simulink model "ACFT11_a_121_flatearth_backup"  (R2026a)
settings: Solver=ode15s  StopTime=10  FixedStep=0.01  MaxStep=0.05  MinStep=1e-4  AbsTol=1e-4
model workspace (MAT data in the model file):
  op11 : opcond.OperatingPoint (value not decoded)
  op_trim1 : opcond.OperatingReport (value not decoded)
  op_trim12 : opcond.OperatingReport (value not decoded)
  op_trim15 : opcond.OperatingReport (value not decoded)
  op_trim16 : opcond.OperatingReport (value not decoded)
  op_trim17 : opcond.OperatingReport (value not decoded)
  op_trim18 : opcond.OperatingReport (value not decoded)
  op_trim2 : opcond.OperatingReport (value not decoded)
  op_trim20 : opcond.OperatingReport (value not decoded)
  op_trim21 : opcond.OperatingReport (value not decoded)
  op_trim22 : opcond.OperatingReport (value not decoded)
  op_trim23 : opcond.OperatingReport (value not decoded)
  op_trim24 : opcond.OperatingReport (value not decoded)
  op_trim25 : opcond.OperatingReport (value not decoded)
  op_trim29 : opcond.OperatingReport (value not decoded)
  op_trim3 : opcond.OperatingReport (value not decoded)
  op_trim30 : opcond.OperatingReport (value not decoded)
  op_trim4 : opcond.OperatingReport (value not decoded)
  op_trim40 : opcond.OperatingReport (value not decoded)
  op_trim42 : opcond.OperatingReport (value not decoded)
  op_trim5 : opcond.OperatingReport (value not decoded)
  op_trim50 : opcond.OperatingReport (value not decoded)
  op_trim7 : opcond.OperatingReport (value not decoded)
  op_trim9 : opcond.OperatingReport (value not decoded)
values from neighbouring files (symbols this model uses):
  b = min(1, 2*(1-frac))    [export_kml.m]    (also in flight_hud.m = chaseBack; inertiatensor62.m = 9.05; setup_bfl_analysis.m = 9.05; setup_fcs_sim.m = 9.05)
  c = bar_colors{min(k,numel(bar_colors))}    [analyze_bfl.m]    (also in ecef_eom_fcn.m = w_eb_b(3); inertiatensor62.m = 15.55; optimize_indi_gains.m = 15.55; restore_normal_fcs.m = 15.55)
  CL_AlphaDot = 0    [inertiatensor62.m]    (also in setup_bfl_analysis.m; setup_fcs_sim.m; setup_takeoff_fcs.m)
  Cm_AlphaDot = 0    [inertiatensor62.m]    (also in setup_bfl_analysis.m; setup_fcs_sim.m; setup_takeoff_fcs.m)
  F = convhull(pts)    [Visualization_Takeoff2.m]    (also in attitude_ribbon.m = {[1 2 3],[1 4 2],[1 4 3],[4 5 1]})
  FCS_aerospike_thrust = 250000.0    (= 250000)    [fcs_params.m]
  FCS_alpha_max = 16.0    (= 16)    [fcs_params.m]
  FCS_bank_max = 35.0    (= 35)    [fcs_params.m]
  FCS_da_max = 20.0    (= 20)    [fcs_params.m]
  FCS_de_max = 25.0    (= 25)    [fcs_params.m]
  FCS_dr_max = 25.0    (= 25)    [fcs_params.m]
  FCS_dt = 0.01    [fcs_params.m]
  FCS_g = 9.80665    [fcs_params.m]
  FCS_Gmin_p = 0.02    [fcs_params.m]
  FCS_Gmin_q = 0.02    [fcs_params.m]
  FCS_Gmin_r = 0.01    [fcs_params.m]
  FCS_h_gnd = 2.24    [fcs_params.m]
  FCS_hdot_max = 30.0    (= 30)    [fcs_params.m]
  FCS_hdot_td = 0.3    [fcs_params.m]
  FCS_Kalpha = 3.0    (= 3)    [fcs_params.m]
  FCS_Kalpha_lim = 2.0    (= 2)    [fcs_params.m]
  FCS_Kbeta = 2.0    (= 2)    [fcs_params.m]
  FCS_Kflare = 1.0    (= 1)    [fcs_params.m]
  FCS_Kgamma = 1.5    [fcs_params.m]
  FCS_Kh = 0.10    (= 0.1)    [fcs_params.m]
  FCS_Knz = 20.0    (= 20)    [fcs_params.m]
  FCS_Kp = 6.0    (= 6)    [fcs_params.m]
  FCS_Kphi = 3.0    (= 3)    [fcs_params.m]
  FCS_Kq = 5.0    (= 5)    [fcs_params.m]
  FCS_Kr = 4.0    (= 4)    [fcs_params.m]
  FCS_Ktheta = 2.0    (= 2)    [fcs_params.m]
  FCS_link_timeout = 1.0    (= 1)    [fcs_params.m]
  FCS_MODE_AUTO = 0    [fcs_params.m]
  FCS_Nfilt = 20.0    (= 20)    [fcs_params.m]
  FCS_Nz_max = 3.0    (= 3)    [fcs_params.m]
  FCS_Nz_min = -1.0    (= -1)    [fcs_params.m]
  FCS_p_max = 40.0    (= 40)    [fcs_params.m]
  FCS_q_max = 15.0    (= 15)    [fcs_params.m]
  FCS_qbar_hi = 6000.0    (= 6000)    [fcs_params.m]
  FCS_qbar_lo = 1000.0    (= 1000)    [fcs_params.m]
  FCS_r_max = 15.0    (= 15)    [fcs_params.m]
  FCS_relight_M_hi = 2.0    (= 2)    [fcs_params.m]
  FCS_relight_M_lo = 0.35    [fcs_params.m]
  FCS_relight_qbar = 3000.0    (= 3000)    [fcs_params.m]
  FCS_stick_detent = 0.03    [fcs_params.m]
  FCS_stick_p_scale = 60.0    (= 60)    [fcs_params.m]
  FCS_stick_q_scale = 15.0    (= 15)    [fcs_params.m]
  FCS_tau_flare = 3.0    (= 3)    [fcs_params.m]
  FCS_TECS_Kep = 0.25    [fcs_params.m]
  FCS_TECS_Ktp = 0.30    (= 0.3)    [fcs_params.m]
  FCS_theta_climb = 12.0    (= 12)    [fcs_params.m]
  FCS_theta_max = 30.0    (= 30)    [fcs_params.m]
  FCS_theta_min = -20.0    (= -20)    [fcs_params.m]
  FCS_theta_trim = 0.0    (= 0)    [fcs_params.m]
  FCS_thr_max = 1.0    (= 1)    [fcs_params.m]
  FCS_thr_min = 0.0    (= 0)    [fcs_params.m]
  FCS_thr_trim = 0.50    (= 0.5)    [fcs_params.m]
  FCS_V_rotate = 94.0    (= 94)    [fcs_params.m]
  FCS_Vmin = 60.0    (= 60)    [fcs_params.m]
  FF_rates = [0.0,              2.5,              5.0,             73.0,             78.0,              0.5]    [fcs_params.m]
  g = @(n,d) i_basevar(n,d)    [analyze_control_authority.m]    (also in export_kml.m = 1 - abs(2*frac-1); inertiatensor62.m = 9.80665; setup_bfl_analysis.m = 9.80665; setup_fcs_sim.m = 9.80665)
  GS_Gp_tab = Cl_da * (S*b/Ixx)    [setup_gschedule.m]
  GS_Gq_tab = Cm_de * (S*c/Iyy)    [setup_gschedule.m]
  GS_Gr_tab = Cn_dr * (S*b/Izz)    [setup_gschedule.m]
  MASS_fuel_total = MASS_full - MASS_empty - MASS_orbiter    (= 14700)    [fcs_params.m]
  q = q/norm(q)    [build_ecef_x0.m]    (also in ecef_eom_fcn.m = state(7:10); ecef_out_fcn.m = state(7:10); setup_ecef.m; test_ecef_eom.m = state(7:10))
  r = [0;diff(xc)]/0.1    [analyze_control_authority.m]    (also in ecef_eom_fcn.m = sqrt(r_e(1)^2+r_e(2)^2+r_e(3)^2); ecef_weight_body.m = sqrt(x^2 + y^2 + z^2); export_kml.m = min(1, 2*frac); test_ecef_eom.m = sqrt(r_e(1)^2+r_e(2)^2+r_e(3)^2))
  S = {'\delta_e',DE,lim.de,'b'; '\delta_a',DA,lim.da,[0 .6 0]; '\delta_r',DR,lim.dr,[.85 .3 .1]}    [analyze_control_authority.m]    (also in attitude_ribbon.m = load(char(src)); build_ecef_x0.m = sqrt(1+C(3,3)-C(1,1)-C(2,2))*2; export_kml.m = load(char(src)); flight_hud.m = load(char(src)))
  s = A.surfaces(i)    [analyze_control_authority.m]    (also in setup_propulsion.m = [s, sprintf(')
  y_cg = 0    [inertiatensor62.m]    (also in setup_bfl_analysis.m; setup_fcs_sim.m; setup_takeoff_fcs.m)
  z_cg = 0.0    (= 0)    [inertiatensor62.m]    (also in setup_bfl_analysis.m; setup_fcs_sim.m; setup_takeoff_fcs.m)
undefined symbols (not defined in the file or in its folder): deg, DiscIntNeverNeededParam, EqM, GS_alpha_cl, GS_alpha_cm, GS_alpha_cn, GS_mach_cl, GS_mach_cm, GS_mach_cn, MIL, Moderate, rad
libraries: aerolibconvert2 x21, simulink x7, aerolibfltsims x3, aerolibwind2 x3, aerolibanim x1, aerolibatmos2 x1, shareddyn x1, aerolibobsolete x1
(part 4 of 4)

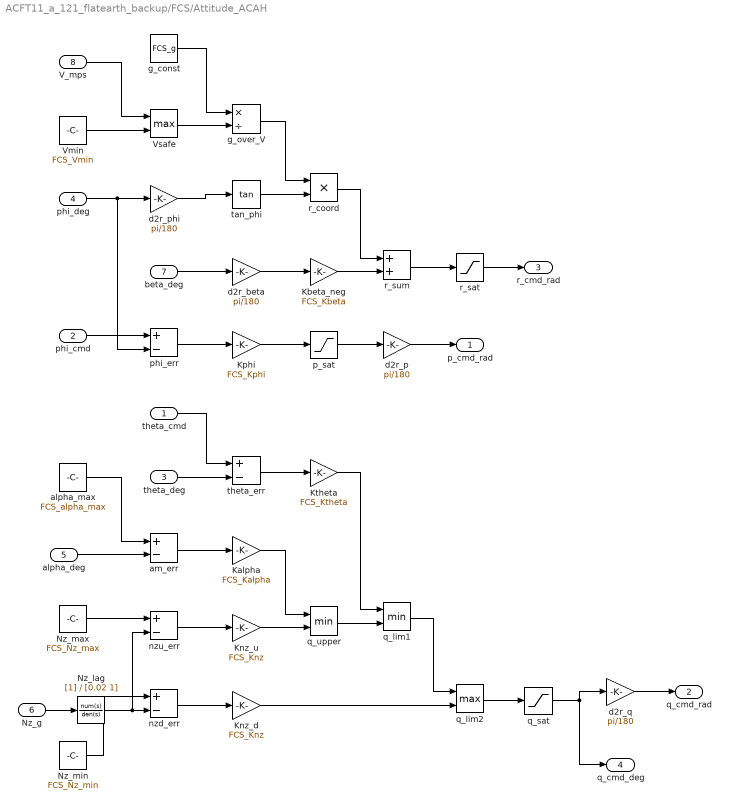
== system ACFT11_a_121_flatearth_backup/FCS/Attitude_ACAH ==
  theta_cmd : Inport
  phi_cmd : Inport  Port=2
  theta_deg : Inport  Port=3
  phi_deg : Inport  Port=4
  alpha_deg : Inport  Port=5
  Nz_g : Inport  Port=6
  beta_deg : Inport  Port=7
  V_mps : Inport  Port=8
  Kalpha : Gain  Gain=FCS_Kalpha
  Kbeta_neg : Gain  Gain=FCS_Kbeta
  Knz_d : Gain  Gain=FCS_Knz
  Knz_u : Gain  Gain=FCS_Knz
  Kphi : Gain  Gain=FCS_Kphi
  Ktheta : Gain  Gain=FCS_Ktheta
  Nz_lag : TransferFcn  Denominator=[0.02 1]
  Nz_max : Constant  Value=FCS_Nz_max
  Nz_min : Constant  Value=FCS_Nz_min
  Vmin : Constant  Value=FCS_Vmin
  Vsafe : MinMax  Function=max  Inputs=2
  alpha_max : Constant  Value=FCS_alpha_max
  am_err : Sum  Inputs=+-
  d2r_beta : Gain  Gain=pi/180
  d2r_p : Gain  Gain=pi/180
  d2r_phi : Gain  Gain=pi/180
  d2r_q : Gain  Gain=pi/180
  g_const : Constant  Value=FCS_g
  g_over_V : Product  Inputs=*/
  nzd_err : Sum  Inputs=+-
  nzu_err : Sum  Inputs=+-
  p_sat : Saturate  UpperLimit=FCS_p_max  LowerLimit=-FCS_p_max
  phi_err : Sum  Inputs=+-
  q_lim1 : MinMax  Inputs=2
  q_lim2 : MinMax  Function=max  Inputs=2
  q_sat : Saturate  UpperLimit=FCS_q_max  LowerLimit=-FCS_q_max
  q_upper : MinMax  Inputs=2
  r_coord : Product  Inputs=**
  r_sat : Saturate  UpperLimit=FCS_r_max*pi/180  LowerLimit=-FCS_r_max*pi/180
  r_sum : Sum
  tan_phi : Trigonometry  Operator=tan
  theta_err : Sum  Inputs=+-
  p_cmd_rad : Outport
  q_cmd_rad : Outport  Port=2
  r_cmd_rad : Outport  Port=3
  q_cmd_deg : Outport  Port=4
  wires:
  r_sat/1 -> r_cmd_rad/1
  r_sum/1 -> r_sat/1
  Kbeta_neg/1 -> r_sum/2
  r_coord/1 -> r_sum/1
  d2r_beta/1 -> Kbeta_neg/1
  beta_deg/1 -> d2r_beta/1
  tan_phi/1 -> r_coord/2
  g_over_V/1 -> r_coord/1
  Vsafe/1 -> g_over_V/2
  g_const/1 -> g_over_V/1
  Vmin/1 -> Vsafe/2
  V_mps/1 -> Vsafe/1
  d2r_phi/1 -> tan_phi/1
  d2r_p/1 -> p_cmd_rad/1
  p_sat/1 -> d2r_p/1
  Kphi/1 -> p_sat/1
  phi_err/1 -> Kphi/1
  phi_deg/1 -> phi_err/2, d2r_phi/1
  phi_cmd/1 -> phi_err/1
  d2r_q/1 -> q_cmd_rad/1
  q_sat/1 -> q_cmd_deg/1, d2r_q/1
  q_lim2/1 -> q_sat/1
  Knz_d/1 -> q_lim2/2
  q_lim1/1 -> q_lim2/1
  q_upper/1 -> q_lim1/2
  Ktheta/1 -> q_lim1/1
  Knz_u/1 -> q_upper/2
  Kalpha/1 -> q_upper/1
  nzd_err/1 -> Knz_d/1
  Nz_min/1 -> nzd_err/1
  nzu_err/1 -> Knz_u/1
  Nz_max/1 -> nzu_err/1
  am_err/1 -> Kalpha/1
  alpha_deg/1 -> am_err/2
  alpha_max/1 -> am_err/1
  theta_err/1 -> Ktheta/1
  theta_deg/1 -> theta_err/2
  theta_cmd/1 -> theta_err/1
  Nz_g/1 -> Nz_lag/1
  Nz_lag/1 -> nzu_err/2, nzd_err/2

== system ACFT11_a_121_flatearth_backup/FCS/HeadingHold ==
  track : Inport
  psi_cmd : Inport  Port=2
  V : Inport  Port=3
  qbar : Inport  Port=4
  L1law : MATLAB Function  TreatAsAtomicUnit=on
  bank_sat : Saturate  UpperLimit=FCS_bank_max  LowerLimit=-FCS_bank_max
  phi_cmd : Outport
  wires:
  L1law/1(phi) -> bank_sat/1
  V/1 -> L1law/3(V)
  track/1 -> L1law/2(track)
  psi_cmd/1 -> L1law/1(psi_cmd)
  bank_sat/1 -> phi_cmd/1
  qbar/1 -> L1law/4(qbar)

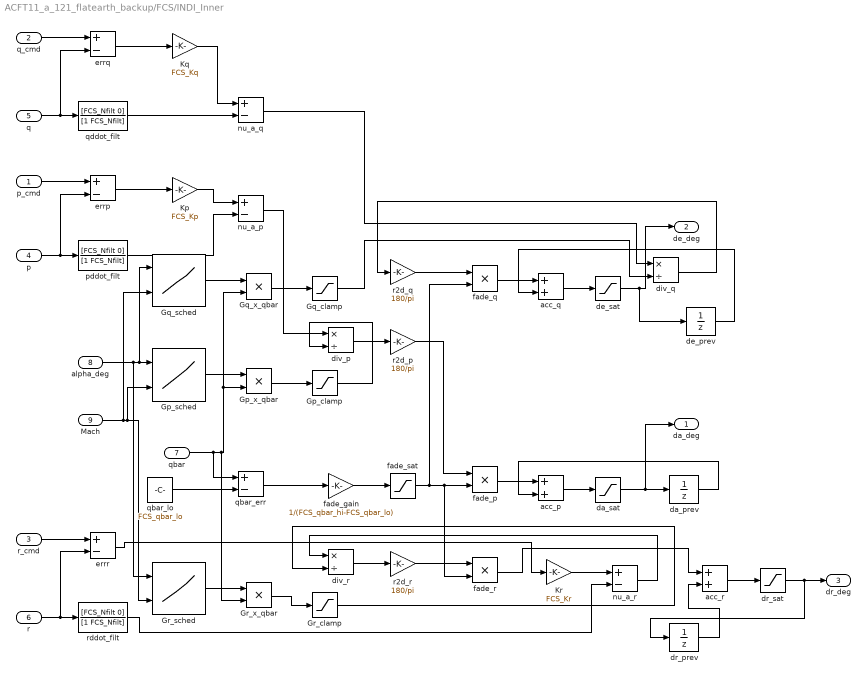
== system ACFT11_a_121_flatearth_backup/FCS/INDI_Inner ==
  p_cmd : Inport
  q_cmd : Inport  Port=2
  r_cmd : Inport  Port=3
  p : Inport  Port=4
  q : Inport  Port=5
  r : Inport  Port=6
  qbar : Inport  Port=7
  alpha_deg : Inport  Port=8
  Mach : Inport  Port=9
  Gp_clamp : Saturate  UpperLimit=-FCS_Gmin_p  LowerLimit=-1e6
  Gp_sched : Lookup_n-D  BreakpointsForDimension1=GS_alpha_cl  BreakpointsForDimension2=GS_mach_cl  Table=GS_Gp_tab  ExtrapMethod=Clip  InternalRulePriority=Speed  RndMeth=Simplest
      settings: InputPortMap=u0,u1
  Gp_x_qbar : Product
  Gq_clamp : Saturate  UpperLimit=-FCS_Gmin_q  LowerLimit=-1e6
  Gq_sched : Lookup_n-D  BreakpointsForDimension1=GS_alpha_cm  BreakpointsForDimension2=GS_mach_cm  Table=GS_Gq_tab  ExtrapMethod=Clip  InternalRulePriority=Speed  RndMeth=Simplest
      settings: InputPortMap=u0,u1
  Gq_x_qbar : Product
  Gr_clamp : Saturate  UpperLimit=-FCS_Gmin_r  LowerLimit=-1e6
  Gr_sched : Lookup_n-D  BreakpointsForDimension1=GS_alpha_cn  BreakpointsForDimension2=GS_mach_cn  Table=GS_Gr_tab  ExtrapMethod=Clip  InternalRulePriority=Speed  RndMeth=Simplest
      settings: InputPortMap=u0,u1
  Gr_x_qbar : Product
  Kp : Gain  Gain=FCS_Kp
  Kq : Gain  Gain=FCS_Kq
  Kr : Gain  Gain=FCS_Kr
  acc_p : Sum
  acc_q : Sum
  acc_r : Sum
  da_prev : UnitDelay  SampleTime=FCS_dt
  da_sat : Saturate  UpperLimit=FCS_da_max  LowerLimit=-FCS_da_max
  de_prev : UnitDelay  SampleTime=FCS_dt
  de_sat : Saturate  UpperLimit=FCS_de_max  LowerLimit=-FCS_de_max
  div_p : Product  Inputs=*/
  div_q : Product  Inputs=*/
  div_r : Product  Inputs=*/
  dr_prev : UnitDelay  SampleTime=FCS_dt
  dr_sat : Saturate  UpperLimit=FCS_dr_max  LowerLimit=-FCS_dr_max
  errp : Sum  Inputs=+-
  errq : Sum  Inputs=+-
  errr : Sum  Inputs=+-
  fade_gain : Gain  Gain=1/(FCS_qbar_hi-FCS_qbar_lo)
  fade_p : Product  Inputs=**
  fade_q : Product  Inputs=**
  fade_r : Product  Inputs=**
  fade_sat : Saturate  UpperLimit=1  LowerLimit=0
  nu_a_p : Sum  Inputs=+-
  nu_a_q : Sum  Inputs=+-
  nu_a_r : Sum  Inputs=+-
  pddot_filt : TransferFcn  Numerator=[FCS_Nfilt 0]  Denominator=[1 FCS_Nfilt]
  qbar_err : Sum  Inputs=+-
  qbar_lo : Constant  Value=FCS_qbar_lo
  qddot_filt : TransferFcn  Numerator=[FCS_Nfilt 0]  Denominator=[1 FCS_Nfilt]
  r2d_p : Gain  Gain=180/pi
  r2d_q : Gain  Gain=180/pi
  r2d_r : Gain  Gain=180/pi
  rddot_filt : TransferFcn  Numerator=[FCS_Nfilt 0]  Denominator=[1 FCS_Nfilt]
  da_deg : Outport
  de_deg : Outport  Port=2
  dr_deg : Outport  Port=3
  wires:
  r2d_r/1 -> fade_r/1
  fade_p/1 -> acc_p/1
  r2d_p/1 -> fade_p/1
  fade_q/1 -> acc_q/1
  fade_sat/1 -> fade_p/2, fade_r/2, fade_q/2
  r2d_q/1 -> fade_q/1
  fade_gain/1 -> fade_sat/1
  qbar_err/1 -> fade_gain/1
  qbar_lo/1 -> qbar_err/2
  da_sat/1 -> da_prev/1, da_deg/1
  acc_p/1 -> da_sat/1
  da_prev/1 -> acc_p/2
  div_p/1 -> r2d_p/1
  nu_a_p/1 -> div_p/1
  pddot_filt/1 -> nu_a_p/2
  Kp/1 -> nu_a_p/1
  errp/1 -> Kp/1
  p/1 -> errp/2, pddot_filt/1
  p_cmd/1 -> errp/1
  qddot_filt/1 -> nu_a_q/2
  Kq/1 -> nu_a_q/1
  errq/1 -> Kq/1
  q/1 -> errq/2, qddot_filt/1
  q_cmd/1 -> errq/1
  acc_q/1 -> de_sat/1
  r_cmd/1 -> errr/1
  r/1 -> rddot_filt/1, errr/2
  div_r/1 -> r2d_r/1
  Gr_x_qbar/1 -> Gr_clamp/1
  Gr_sched/1 -> Gr_x_qbar/1
  Gp_x_qbar/1 -> Gp_clamp/1
  Gp_sched/1 -> Gp_x_qbar/1
  Gq_x_qbar/1 -> Gq_clamp/1
  Gq_sched/1 -> Gq_x_qbar/1
  Mach/1 -> Gr_sched/2, Gp_sched/2, Gq_sched/2
  alpha_deg/1 -> Gq_sched/1, Gp_sched/1, Gr_sched/1
  dr_sat/1 -> dr_prev/1, dr_deg/1
  acc_r/1 -> dr_sat/1
  dr_prev/1 -> acc_r/2
  Gr_clamp/1 -> div_r/2
  nu_a_r/1 -> div_r/1
  rddot_filt/1 -> nu_a_r/2
  Kr/1 -> nu_a_r/1
  errr/1 -> Kr/1
  de_sat/1 -> de_prev/1, de_deg/1
  Gq_clamp/1 -> div_q/2
  qbar/1 -> Gp_x_qbar/2, Gq_x_qbar/2, Gr_x_qbar/2, qbar_err/1
  nu_a_q/1 -> div_q/1
  div_q/1 -> r2d_q/1
  de_prev/1 -> acc_q/2
  Gp_clamp/1 -> div_p/2
  fade_r/1 -> acc_r/1

== system ACFT11_a_121_flatearth_backup/FCS/ModeManager ==
  RC_mode : Inport
  RC_cmd_age : Inport  Port=2
  theta_TECS : Inport  Port=3
  theta_ref : Inport  Port=4
  phi_hdg : Inport  Port=5
  phi_ref : Inport  Port=6
  AUTO : Constant  Value=FCS_MODE_AUTO
  link_lost : simulink/Logic and Bit Operations/Compare To Constant  relop=>  const=FCS_link_timeout  OutDataTypeStr=boolean
  mode_sw : Switch  Threshold=0.5  SaturateOnIntegerOverflow=off  InputSameDT=off
  phi_sw : Switch  Threshold=0.5  SaturateOnIntegerOverflow=off  InputSameDT=off
  theta_sw : Switch  Threshold=0.5  SaturateOnIntegerOverflow=off  InputSameDT=off
  theta_cmd_sel : Outport
  phi_cmd_sel : Outport  Port=2
  mode_eff : Outport  Port=3
  wires:
  phi_sw/1 -> phi_cmd_sel/1
  phi_hdg/1 -> phi_sw/3
  phi_ref/1 -> phi_sw/1
  theta_sw/1 -> theta_cmd_sel/1
  theta_TECS/1 -> theta_sw/3
  theta_ref/1 -> theta_sw/1
  mode_sw/1 -> mode_eff/1, phi_sw/2, theta_sw/2
  RC_mode/1 -> mode_sw/3
  link_lost/1 -> mode_sw/2
  AUTO/1 -> mode_sw/1
  RC_cmd_age/1 -> link_lost/1

== system ACFT11_a_121_flatearth_backup/FCS/Pilot_RCAH ==
  RC_pitch : Inport
  RC_roll : Inport  Port=2
  mode_eff : Inport  Port=3
  theta_deg : Inport  Port=4
  phi_deg : Inport  Port=5
  dz_pitch : DeadZone  LowerValue=-FCS_stick_detent  UpperValue=FCS_stick_detent
  dz_roll : DeadZone  LowerValue=-FCS_stick_detent  UpperValue=FCS_stick_detent
  phi_ref_int : DiscreteIntegrator  gainval=1  ExternalReset=level  InitialConditionSource=external  SampleTime=FCS_dt  LimitOutput=on  UpperSaturationLimit=FCS_bank_max  LowerSaturationLimit=-FCS_bank_max  ICPrevOutput=DiscIntNeverNeededParam  ICPrevScaledInput=DiscIntNeverNeededParam
  reset_auto : simulink/Logic and Bit Operations/Compare To Constant  relop=<  const=0.5  OutDataTypeStr=boolean
  sc_pitch : Gain  Gain=FCS_stick_q_scale
  sc_roll : Gain  Gain=FCS_stick_p_scale
  theta_ref_int : DiscreteIntegrator  gainval=1  ExternalReset=level  InitialConditionSource=external  SampleTime=FCS_dt  LimitOutput=on  UpperSaturationLimit=FCS_theta_max  LowerSaturationLimit=FCS_theta_min  ICPrevOutput=DiscIntNeverNeededParam  ICPrevScaledInput=DiscIntNeverNeededParam
  theta_ref : Outport
  phi_ref : Outport  Port=2
  wires:
  phi_ref_int/1 -> phi_ref/1
  phi_deg/1 -> phi_ref_int/3
  sc_roll/1 -> phi_ref_int/1
  dz_roll/1 -> sc_roll/1
  RC_roll/1 -> dz_roll/1
  theta_ref_int/1 -> theta_ref/1
  theta_deg/1 -> theta_ref_int/3
  reset_auto/1 -> theta_ref_int/2, phi_ref_int/2
  sc_pitch/1 -> theta_ref_int/1
  dz_pitch/1 -> sc_pitch/1
  RC_pitch/1 -> dz_pitch/1
  mode_eff/1 -> reset_auto/1

== system ACFT11_a_121_flatearth_backup/FCS/TECS ==
  V : Inport
  alt : Inport  Port=2
  Vz : Inport  Port=3
  V_cmd : Inport  Port=4
  h_cmd : Inport  Port=5
  Kep : Gain  Gain=FCS_TECS_Kep
  Kh : Gain  Gain=FCS_Kh
  Ktp : Gain  Gain=FCS_TECS_Ktp
  SPE : Sum  Inputs=+-
  Verr : Sum  Inputs=+-
  eBal : Sum  Inputs=+-
  eThr : Sum
  hdot_dem : Saturate  UpperLimit=FCS_hdot_max  LowerLimit=-FCS_hdot_max
  herr : Sum  Inputs=+-
  pitch_int : DiscreteIntegrator  gainval=FCS_TECS_Kei  InitialCondition=FCS_theta_trim  SampleTime=FCS_dt  LimitOutput=on  UpperSaturationLimit=FCS_theta_max  LowerSaturationLimit=FCS_theta_min  ICPrevOutput=DiscIntNeverNeededParam  ICPrevScaledInput=DiscIntNeverNeededParam
  th_out : Saturate  UpperLimit=FCS_theta_max  LowerLimit=FCS_theta_min
  th_sum : Sum
  thr_int : DiscreteIntegrator  gainval=FCS_TECS_Kti  InitialCondition=FCS_thr_trim  SampleTime=FCS_dt  LimitOutput=on  UpperSaturationLimit=FCS_thr_max  LowerSaturationLimit=FCS_thr_min  ICPrevOutput=DiscIntNeverNeededParam  ICPrevScaledInput=DiscIntNeverNeededParam
  thr_out : Saturate  UpperLimit=FCS_thr_max  LowerLimit=FCS_thr_min
  thr_sum : Sum
  theta_cmd : Outport
  Throttle : Outport  Port=2
  wires:
  h_cmd/1 -> herr/1
  V_cmd/1 -> Verr/1
  V/1 -> Verr/2
  alt/1 -> herr/2
  herr/1 -> Kh/1
  Kh/1 -> hdot_dem/1
  hdot_dem/1 -> SPE/1
  Vz/1 -> SPE/2
  SPE/1 -> eBal/1, eThr/1
  Verr/1 -> eBal/2, eThr/2
  eThr/1 -> thr_int/1, Ktp/1
  Ktp/1 -> thr_sum/1
  thr_int/1 -> thr_sum/2
  thr_sum/1 -> thr_out/1
  thr_out/1 -> Throttle/1
  eBal/1 -> pitch_int/1, Kep/1
  Kep/1 -> th_sum/1
  pitch_int/1 -> th_sum/2
  th_sum/1 -> th_out/1
  th_out/1 -> theta_cmd/1

== system ACFT11_a_121_flatearth_backup/EqM/BodyRates/CrossProduct ==
  A : Inport
  B : Inport  Port=2
  Add : Sum  Inputs=+-
  Demux : Demux  Outputs=3
  Demux1 : Demux  Outputs=3
  Mux : Mux  Inputs=3
  Mux1 : Mux  Inputs=3
  Product{,1..5} (6 alike) : Product
  C : Outport
  wires:
  Add/1 -> C/1  "A X B"
  Product2/1 -> Mux/3
  Product/1 -> Mux/1
  Demux/1 -> Product2/1, Product4/1
  Demux1/2 -> Product2/2, Product3/2
  Demux/3 -> Product1/1, Product3/1
  B/1 -> Demux1/1
  Mux1/1 -> Add/2
  Demux/2 -> Product/1, Product5/1
  A/1 -> Demux/1
  Product3/1 -> Mux1/1
  Demux1/1 -> Product1/2, Product5/2
  Mux/1 -> Add/1
  Product5/1 -> Mux1/3
  Product1/1 -> Mux/2
  Demux1/3 -> Product/2, Product4/2
  Product4/1 -> Mux1/2

== system ACFT11_a_121_flatearth_backup/EqM/BodyVelocities/CrossProduct ==
  A : Inport
  B : Inport  Port=2
  Add : Sum  Inputs=+-
  Demux : Demux  Outputs=3
  Demux1 : Demux  Outputs=3
  Mux : Mux  Inputs=3
  Mux1 : Mux  Inputs=3
  Product{,1..5} (6 alike) : Product
  C : Outport
  wires:
  Add/1 -> C/1  "A X B"
  Product2/1 -> Mux/3
  Product/1 -> Mux/1
  Demux/1 -> Product2/1, Product4/1
  Demux1/2 -> Product2/2, Product3/2
  Demux/3 -> Product1/1, Product3/1
  B/1 -> Demux1/1
  Mux1/1 -> Add/2
  Demux/2 -> Product/1, Product5/1
  A/1 -> Demux/1
  Product3/1 -> Mux1/1
  Demux1/1 -> Product1/2, Product5/2
  Mux/1 -> Add/1
  Product5/1 -> Mux1/3
  Product1/1 -> Mux/2
  Demux1/3 -> Product/2, Product4/2
  Product4/1 -> Mux1/2

== system ACFT11_a_121_flatearth_backup/EqM/EulerAngles/EulerRates ==
  BodyRates_radps : Inport
  EulerAngles_rad : Inport  Port=2
  Abs : Abs  SaturateOnIntegerOverflow=off
  Constant : Constant  Value=0.001
  Demux : Demux  Outputs=3
  Mux : Mux  Inputs=3
  Mux1 : Mux  Inputs=3
  Mux2 : Mux  Inputs=3
  Product : Product
  Relay : Relay  OnSwitchValue=.001  OffSwitchValue=0  OnOutputValue=0  OffOutputValue=1
  Sign : Signum
  Switch : Switch  Criteria=u2 > Threshold  Threshold=0.5  SaturateOnIntegerOverflow=off  InputSameDT=off
  Trigonometric Function : Trigonometry  Operator=sincos
  phidot_radps2 : Fcn  Expr=u(1)+u(2)*u(4)*(u(5)/u(8))+u(3)*u(7)*(u(5)/u(8))
  psidot_radps2 : Fcn  Expr=(u(2)*u(4)+u(3)*u(7))/u(8)
  thetadot_radps2 : Fcn  Expr=u(2)*u(7)-u(3)*u(4)
  EulerRates_radsps2 : Outport
  wires:
  Mux1/1 -> Mux/3
  Trigonometric Function/1 -> Mux/2
  Demux/3 -> Mux1/3
  Constant/1 -> Product/1
  Sign/1 -> Product/2
  Switch/1 -> Mux1/2
  Demux/2 -> Switch/3, Abs/1, Sign/1
  Mux2/1 -> EulerRates_radsps2/1
  psidot_radps2/1 -> Mux2/3
  Product/1 -> Switch/1
  Abs/1 -> Relay/1
  thetadot_radps2/1 -> Mux2/2
  phidot_radps2/1 -> Mux2/1
  BodyRates_radps/1 -> Mux/1
  Relay/1 -> Switch/2
  Demux/1 -> Mux1/1
  Trigonometric Function/2 -> Demux/1
  EulerAngles_rad/1 -> Trigonometric Function/1
  Mux/1 -> psidot_radps2/1, thetadot_radps2/1, phidot_radps2/1

== system ACFT11_a_121_flatearth_backup/EqM/EulerAngles/LBE_rotation ==
  note: LBE
  EulerAngles_rad : Inport
  Math Function : Math  Operator=transpose  SignedPower=on
  Mux : Mux  Inputs=2
  Mux2 : Mux  Inputs=9
  Reshape : Reshape  OutputDimensionality=Customize  OutputDimensions=[3,3]
  Trigonometric Function : Trigonometry  Operator=sincos
  phidot_radps1 : Fcn  Expr=u(1)*u(2)*u(6) - u(4)*u(3)
  phidot_radps2 : Fcn  Expr=u(5)*u(6)
  phidot_radps3 : Fcn  Expr=u(6)*u(2)*u(4) + u(1)*u(3)
  phidot_radps4 : Fcn  Expr=u(5)*u(3)
  phidot_radps5 : Fcn  Expr=u(1)*u(2)*u(3) + u(4)*u(6)
  phidot_radps6 : Fcn  Expr=u(4)*u(2)*u(3) -u(1)*u(6)
  phidot_radps7 : Fcn  Expr=-u(2)
  phidot_radps8 : Fcn  Expr=u(1)*u(5)
  phidot_radps9 : Fcn  Expr=u(4)*u(5)
  LBE : Outport
  wires:
  phidot_radps9/1 -> Mux2/9
  phidot_radps8/1 -> Mux2/8
  phidot_radps7/1 -> Mux2/7
  phidot_radps5/1 -> Mux2/5
  phidot_radps6/1 -> Mux2/6
  Mux/1 -> phidot_radps4/1, phidot_radps5/1, phidot_radps6/1, phidot_radps7/1, phidot_radps8/1, phidot_radps9/1, phidot_radps2/1, phidot_radps1/1, phidot_radps3/1
  Trigonometric Function/1 -> Mux/1
  phidot_radps1/1 -> Mux2/2
  phidot_radps2/1 -> Mux2/1
  phidot_radps4/1 -> Mux2/4
  phidot_radps3/1 -> Mux2/3
  Math Function/1 -> LBE/1
  Reshape/1 -> Math Function/1
  Mux2/1 -> Reshape/1
  Trigonometric Function/2 -> Mux/2
  EulerAngles_rad/1 -> Trigonometric Function/1

== matlab function ACFT11_a_121_flatearth_backup/RTB_Guidance ==
  data: pos_NED input; range_home output; bearing_home output; xtrack_err output; along_track output; gs_alt_cmd output; loc_hdg_cmd output
function [range_home, bearing_home, xtrack_err, along_track, gs_alt_cmd, loc_hdg_cmd] = RTB_Guidance(pos_NED)
%#codegen
rwy_N = 0.0; rwy_E = 0.0; rwy_hdg = 180.0;
gs_steep = 4.0; gs_shallow = 2.5; R_break = 3000.0; K_loc = 0.02; loc_max = 20.0;
dN = rwy_N - pos_NED(1); dE = rwy_E - pos_NED(2);
range_home = sqrt(dN*dN + dE*dE);
psi = atan2(dE, dN) * 180/pi;
if psi < 0, psi = psi + 360; end
bearing_home = psi;
rwy_rad = rwy_hdg * pi / 180;
uN = cos(rwy_rad); uE = sin(rwy_rad);
relN = pos_NED(1) - rwy_N; relE = pos_NED(2) - rwy_E;
along_track = -(relN * uN + relE * uE);
xtrack_err = -relN * uE + relE * uN;
h_break = R_break * tand(gs_shallow);
if along_track <= R_break
    gs_alt_cmd = along_track * tand(gs_shallow);
else
    gs_alt_cmd = h_break + (along_track - R_break) * tand(gs_steep);
end
if gs_alt_cmd < 0, gs_alt_cmd = 0; end
loc_corr = -K_loc * xtrack_err;
if loc_corr > loc_max, loc_corr = loc_max; end
if loc_corr < -loc_max, loc_corr = -loc_max; end
loc_hdg_cmd = rwy_hdg + loc_corr;
if loc_hdg_cmd < 0, loc_hdg_cmd = loc_hdg_cmd + 360; end
if loc_hdg_cmd >= 360, loc_hdg_cmd = loc_hdg_cmd - 360; end
end

== matlab function ACFT11_a_121_flatearth_backup/Landing Gear/LandingGear_FCN ==
  data: EulerAngles_rad input; GndForces output; VB_mps input; BodyRates_radps input; pos_NED_m input; mass_kg input; N_total output; N_gears output; mu_cmd input
function [GndForces, N_total, N_gears] = LandingGear_FCN(EulerAngles_rad, VB_mps, BodyRates_radps, pos_NED_m, mass_kg, mu_cmd)
%#codegen
% Landing gear: spring-damper, one-sided damper (no tension).
% Body frame: x-fwd, y-right, z-DOWN.
% Auto-generated by setup_landing_gear.m
%   mass_kg = 28500  |  delta_static = 0.0800 m  |  zeta = 5.0
% --- Gear arm vectors from CG [x_fwd, y_right, z_down] m -----------
r_NLG   = [6.7600; 0.0000; 2.5580];
r_MLG_L = [-1.0150; -2.3000; 2.2860];
r_MLG_R = [-1.0150; 2.3000; 2.2860];
% --- Spring-damper constants ----------------------------------------
k_NLG = 456100;   c_NLG = 411900;
k_MLG = 1518800;   c_MLG = 1371800;
mu    = mu_cmd;   % 0.03 rolling | 0.3 full brakes (from FCS)
% --- Unpack states --------------------------------------------------
phi=EulerAngles_rad(1); theta=EulerAngles_rad(2); psi=EulerAngles_rad(3);
cph=cos(phi); sph=sin(phi); cth=cos(theta); sth=sin(theta);
cps=cos(psi); sps=sin(psi);
R_BE=[cth*cps, sph*sth*cps-cph*sps, cph*sth*cps+sph*sps;
      cth*sps, sph*sth*sps+cph*cps, cph*sth*sps-sph*cps;
     -sth,     sph*cth,              cph*cth];
h_CG = -pos_NED_m(3);   % NED z positive-down; altitude = -z_NED
% --- Gear compressions (positive = wheel penetrating ground) --------
d_NLG   = (R_BE(3,:)*r_NLG)   - h_CG;
d_MLG_L = (R_BE(3,:)*r_MLG_L) - h_CG;
d_MLG_R = (R_BE(3,:)*r_MLG_R) - h_CG;
on_NLG   = double(d_NLG   > 0);
on_MLG_L = double(d_MLG_L > 0);
on_MLG_R = double(d_MLG_R > 0);
% --- Gear-tip velocity in NED (z-component = compression rate) ------
vn_NLG   = R_BE*(VB_mps+cross(BodyRates_radps,r_NLG));
vn_MLG_L = R_BE*(VB_mps+cross(BodyRates_radps,r_MLG_L));
vn_MLG_R = R_BE*(VB_mps+cross(BodyRates_radps,r_MLG_R));
% --- Normal forces (one-sided damper: damping only on compression) --
N_NLG   = max(k_NLG*d_NLG   + c_NLG*max(vn_NLG(3),  0)*on_NLG,   0);
N_MLG_L = max(k_MLG*d_MLG_L + c_MLG*max(vn_MLG_L(3),0)*on_MLG_L, 0);
N_MLG_R = max(k_MLG*d_MLG_R + c_MLG*max(vn_MLG_R(3),0)*on_MLG_R, 0);
N_total = N_NLG + N_MLG_L + N_MLG_R;
N_gears = [N_NLG; N_MLG_L; N_MLG_R];
% --- Friction forces ------------------------------------------------
fwd_hat = R_BE(:,1);
sgn_u   = VB_mps(1)/max(abs(VB_mps(1)),0.01);
FN_NED  = fwd_hat*(-mu*N_NLG  *sgn_u)+[0;0;-N_NLG  ];
FL_NED  = fwd_hat*(-mu*N_MLG_L*sgn_u)+[0;0;-N_MLG_L];
FR_NED  = fwd_hat*(-mu*N_MLG_R*sgn_u)+[0;0;-N_MLG_R];
% --- Transform to body frame, compute moments about CG -------------
Fb = R_BE'*(FN_NED+FL_NED+FR_NED);
Mb = cross(r_NLG,  R_BE'*FN_NED) + ...
     cross(r_MLG_L,R_BE'*FL_NED) + ...
     cross(r_MLG_R,R_BE'*FR_NED);
GndForces = [Fb; Mb];   % [Fx;Fy;Fz;Mx;My;Mz] N / N·m
end

== stateflow chart ACFT11_a_121_flatearth_backup/MissionManager ==
  settings: updateMethod=CONTINUOUS
  state GROUND_ROLL
    en: phase=1; law_select=0; thr_cmd=1; q_rot_cmd=0; brake_cmd=FCS_mu_roll; gear_cmd=1; psi_cmd=FCS_runway_hdg; V_cmd=FCS_V_climb; h_cmd=FCS_h_gearsafe; gamma_cmd=0; prop_mode=1; sep_cmd=0;
  state ROTATION
    en: phase=2; law_select=0; thr_cmd=1; q_rot_cmd=FCS_q_rot; brake_cmd=FCS_mu_roll; gear_cmd=1; prop_mode=1;
  state LIFTOFF
    en: phase=3; law_select=3; V_cmd=FCS_V_climb; h_cmd=FCS_h_cruise; gear_cmd=0; thr_cmd=1; q_rot_cmd=0; brake_cmd=0; prop_mode=1;
  state CLIMB1
    en: phase=4; law_select=1; V_cmd=FCS_V_climb; h_cmd=FCS_h_cruise; gear_cmd=0; prop_mode=1;
  state CRUISE1
    en: phase=5; law_select=1; V_cmd=FCS_V_cruise; h_cmd=FCS_h_cruise; prop_mode=1;
  state ACCEL
    en: phase=6; law_select=4; gamma_cmd=0; thr_cmd=1; V_cmd=FCS_V_cruise; h_cmd=FCS_h_cruise; prop_mode=4; sep_cmd=0;
  state ZOOM
    en: phase=7; law_select=4; gamma_cmd=FCS_gamma_zoom; thr_cmd=0; prop_mode=3;
  state SEPARATE
    en: phase=8; law_select=4; gamma_cmd=0; thr_cmd=0; prop_mode=0; sep_cmd=1;
  state COAST
    en: phase=18; law_select=4; gamma_cmd=FCS_gamma_coast; thr_cmd=0; prop_mode=0; sep_cmd=0;
  state GLIDE
    en: phase=9; law_select=4; thr_cmd=0; prop_mode=0; sep_cmd=0;
    du: gamma_cmd = glide_gamma_cmd;
    psi_cmd = glide_psi_cmd;
  state RELIGHT
    en: phase=10; law_select=1; V_cmd=FCS_V_cruise; h_cmd=FCS_h_relight; prop_mode=1;
    du: psi_cmd=bearing_home;
  state CRUISE_RTB
    en: phase=11; law_select=1; V_cmd=FCS_V_cruise; h_cmd=FCS_h_cruise; prop_mode=1;
    du: psi_cmd=bearing_home;
  state DESCEND_RTB
    en: phase=12; law_select=1; V_cmd=FCS_V_desc; h_cmd=FCS_h_platform; prop_mode=1;
    du: psi_cmd=loc_hdg_cmd;
  state APPROACH
    en: phase=13; law_select=1; gear_cmd=1; prop_mode=1;
    du: V_cmd = FCS_V_app + (FCS_V_desc - FCS_V_app)/(1 + exp(-(along_track - FCS_v_decel_ref)/600));
    h_cmd = app_h_cmd;
    psi_cmd = loc_hdg_cmd;
  state FLARE
    en: phase=14; law_select=2; thr_cmd=0; brake_cmd=0; gear_cmd=1; prop_mode=5;
  state TOUCHDOWN
    en: phase=15; law_select=0; thr_cmd=0; q_rot_cmd=-2; brake_cmd=FCS_mu_brake; gear_cmd=1; prop_mode=5;
  state ROLLOUT
    en: phase=16; law_select=0; thr_cmd=0; q_rot_cmd=0; brake_cmd=FCS_mu_brake; gear_cmd=1; prop_mode=5;
  state STOPPED
    en: phase=17; law_select=0; thr_cmd=0; q_rot_cmd=0; brake_cmd=FCS_mu_brake; gear_cmd=1; prop_mode=0;
  (default) -> GROUND_ROLL
  GROUND_ROLL -> ROTATION : [V >= Vr]
  ROTATION -> LIFTOFF : [Ngear <= FCS_WoW_thresh || theta >= FCS_theta_LOF]
  LIFTOFF -> CLIMB1 : [V >= FCS_V_climb]
  CLIMB1 -> CRUISE1 : [h >= FCS_h_cruise - 10]
  CRUISE1 -> ACCEL : [after(FCS_t_cruise1, sec)]
  ACCEL -> ZOOM : [Mach >= FCS_M_trans]
  ZOOM -> SEPARATE : [h >= FCS_h_apogee_tgt]
  SEPARATE -> COAST : [after(FCS_t_sep, sec)]
  COAST -> GLIDE : [descending > 0.5 && qbar >= FCS_qbar_glide]
  GLIDE -> RELIGHT : [h <= FCS_h_relight && relight_ok > 0.5]
  RELIGHT -> CRUISE_RTB : [after(FCS_t_relight, sec)]
  CRUISE_RTB -> DESCEND_RTB : [range_home <= FCS_R_capture]
  DESCEND_RTB -> APPROACH : [gs_alt_cmd <= h + FCS_gs_capture_tol && range_home <= FCS_app_capture_R && xtrack_err <= FCS_loc_tol && xtrack_err >= -FCS_loc_tol]
  APPROACH -> FLARE : [h <= FCS_h_flare]
  FLARE -> TOUCHDOWN : [Ngear >= FCS_WoW_thresh]
  TOUCHDOWN -> ROLLOUT : [V <= FCS_V_derotate]
  ROLLOUT -> STOPPED : [V <= FCS_V_stop]
  data: V input double; h input double; Ngear input double; theta input double; Vr input double; begin_descent input double; phase output double; law_select output double; V_cmd output double; h_cmd output double; psi_cmd output double; q_rot_cmd output double; thr_cmd output double; brake_cmd output double; gear_cmd output double; FCS_theta_LOF parameter double; FCS_WoW_thresh parameter double; FCS_h_gearsafe parameter double; FCS_h_cruise parameter double; FCS_h_approach parameter double; FCS_h_flare parameter double; FCS_V_derotate parameter double; FCS_V_stop parameter double; FCS_q_rot parameter double; FCS_V_climb parameter double; FCS_V_cruise parameter double; FCS_V_desc parameter double; FCS_V_app parameter double; FCS_mu_brake parameter double; FCS_mu_roll parameter double; FCS_runway_hdg parameter double; FCS_hdot_appr parameter double; Mach input double; relight_ok input double; range_home input double; bearing_home input double; gamma_cmd output double; prop_mode output double; sep_cmd output double; FCS_M_trans parameter double; FCS_M_target parameter double; FCS_h_apogee_tgt parameter double; FCS_gamma_zoom parameter double; FCS_gamma_glide parameter double; FCS_h_relight parameter double; FCS_R_capture parameter double; FCS_t_cruise1 parameter double; FCS_t_sep parameter double; FCS_t_relight parameter double; FCS_t_burn parameter double; FCS_gamma_glide_shallow parameter double; FCS_gamma_glide_steep parameter double; FCS_gamma_coast parameter double; qbar input double; FCS_qbar_glide parameter double; descending input double; xtrack_err input; along_track input; gs_alt_cmd input; loc_hdg_cmd input; glide_gamma_cmd input; glide_psi_cmd input; app_h_cmd input; FCS_app_capture_R parameter; FCS_gs_capture_tol parameter; FCS_h_platform parameter; FCS_loc_tol parameter; FCS_gs_break parameter; FCS_v_decel_ref parameter

== matlab function ACFT11_a_121_flatearth_backup/Propulsion/PropulsionFCN ==
  data: Mach input; y output; rho_kgpm3 input; Throttle input
function y = PropulsionFCN(Mach, rho_kgpm3, Throttle)
%#codegen
% 2-engine thrust model: Mach x Altitude lookup table.
% Auto-generated by setup_propulsion.m — edit that file, not this.
%   Engines: 2 x 70 kN SL static  |  incidence = -1.8 deg
%   Output: y = [Fx;0;Fz;0;My;0;Thrust_N]  (7x1)
%           y(1:6) = Engine_Forces_and_Moments,  y(7) = Thrust_N
%
% --- Engine constants -----------------------------------------------
n_eng  = 2;
af_rad = 0;   % engine incidence [rad] (alfaf_deg=-1.80)
xf_m   = 0.0000;   % thrust line x-offset from CG [m]
ye_m   = 0.0000;   % lateral distance of EACH engine from centreline [m]
                 %   engines at +ye_m (right) and -ye_m (left)
                 %   symmetric: Mx,Mz cancel; OEI: Mz = +-ye_m*Fx
zf_m   = 0.0800;   % thrust line z-offset from CG [m]
% --- ISA inverse: rho -> altitude [m] ------------------------------
rho0=1.225; T0=288.15; g0=9.80665; R=287.058; L=0.0065;
rho_11=0.3639; T_11=216.65; h_11=11000.0;
rho_c = max(rho_kgpm3, 1e-4);
if rho_c >= rho_11
    T_K   = T0*(rho_c/rho0)^(1.0/4.2561);
    alt_m = (T0-T_K)/L;
else
    T_K   = T_11;
    alt_m = h_11 + log(rho_11/rho_c)*R*T_11/g0;
end
% --- Mach-Altitude thrust table: ONE engine, Throttle = 1 ----------
Mach_bp = [0, 0.1, 0.2, 0.3, 0.4, 0.5, 0.6, 0.7, 0.8];
Alt_bp  = [0, 2000, 4000, 6000, 8000, 10000, 12000];
T_tab   = [70000, 60000, 51000, 43000, 36000, 29500, 23500;
 72000, 62000, 53000, 44500, 37500, 30500, 24500; 
72500, 62500, 53500, 45000, 38000, 31000, 25000;
 71500, 61500, 52500, 44000, 37000, 30200, 24200; 
70000, 60000, 51500, 43000, 36000, 29500, 23500; 
67500, 58000, 49500, 41500, 35000, 28500, 22500;
 63000, 54000, 46000, 38500, 32500, 26500, 21000;
 57000, 49000, 42000, 35000, 29500, 24000, 19000;
 50000, 43000, 37000, 31000, 26000, 21000, 17000];
% --- Bilinear interpolation (clamped at table boundaries) ----------
T_max_1eng = bilerp(Mach_bp, Alt_bp, T_tab, Mach, alt_m);
% --- Total thrust (both engines, throttle scaled) ------------------
Thrust_N = max(0.0, Throttle * double(n_eng) * T_max_1eng);
% --- Engine force/moment decomposition (body frame) ----------------
% Each engine at [xf_m; ±ye_m; zf_m] relative to CG
% Symmetric pair: Mx,Mz cancel; My = 2*(zf*Fx_1 - xf*Fz_1)
T_1  = Thrust_N * 0.5;
Fx_1 = T_1 * cos(af_rad);
Fz_1 = T_1 * sin(af_rad);
Fx   = 2.0 * Fx_1;
Fz   = 2.0 * Fz_1;
My   = 2.0 * (zf_m*Fx_1 - xf_m*Fz_1);
% Pack output: [forces(6); Thrust_N] — Selector blocks split this
y = [Fx; 0.0; Fz; 0.0; My; 0.0; Thrust_N];
end

% ----- Clamped bilinear interpolation (codegen-safe) ---------------
function Tq = bilerp(Mv, Hv, T, M, H)
%BILERP  Bilinear lookup in 2-D table, clamped at boundaries.
%  Mv [1 x nM], Hv [1 x nH], T [nM x nH], M and H scalars.
nM = numel(Mv); nH_= numel(Hv);
Mc = max(Mv(1), min(Mv(nM),  M));
Hc = max(Hv(1), min(Hv(nH_), H));
im = nM - 1;
for ii = 1:nM-1
    if Mc <= Mv(ii+1); im = ii; break; end
end
ih = nH_ - 1;
for ii = 1:nH_-1
    if Hc <= Hv(ii+1); ih = ii; break; end
end
tm = (Mc - Mv(im)) / (Mv(im+1) - Mv(im));
th = (Hc - Hv(ih)) / (Hv(ih+1) - Hv(ih));
Tq = (1-tm)*(1-th)*T(im,  ih  ) + ...
       tm  *(1-th)*T(im+1,ih  ) + ...
     (1-tm)*  th  *T(im,  ih+1) + ...
       tm  *  th  *T(im+1,ih+1);
end

== matlab function ACFT11_a_121_flatearth_backup/Aerospike ==
  data: prop_mode input; F6 output; T_max input; T_aero output
function [F6, T_aero] = AerospikeThrust(prop_mode, T_max)
%#codegen
% Generic SIMPLIFIED aerospike (rocket) thrust model -- PLACEHOLDER VALUES.
% Fixed-magnitude thrust, commanded ON/OFF by prop_mode from the sequencer.
%   ON when prop_mode is PM_AEROSPIKE (3) or PM_AEROSPIKE_AB (4).
% Thrust acts along body +x through the CG (no thrust-vector moment).
% Propellant mass depletion is NOT modelled here (simplification) --
% T_max is the placeholder fixed thrust (FCS_aerospike_thrust, N).
on = (prop_mode >= 2.5) && (prop_mode <= 4.5);   % true for mode 3 or 4
T_aero = T_max * double(on);
F6 = [T_aero; 0.0; 0.0; 0.0; 0.0; 0.0];   % [Fx; Fy; Fz; Mx; My; Mz] body frame
end

== matlab function ACFT11_a_121_flatearth_backup/RCS_ctrl ==
  data: alpha_deg input; F6 output; phi_rad input; beta_deg input; p input; q input; r input; qbar input; h input
function F6 = RCS_ctrl(alpha_deg, phi_rad, beta_deg, p, q, r, qbar, h)
%#codegen
% Exo-atmospheric Reaction Control System attitude hold for the high-altitude coast.
% Holds alpha~0 / wings-level / zero-sideslip with body moments while aero control is
% ineffective (thin air), so the vehicle tracks the velocity vector down instead of
% mushing to huge alpha. Gated to high altitude and faded out as qbar builds, so it
% never fires on the ground / in dense air -- the aero surfaces take over below.
Ixx=74848; Iyy=288344; Izz=390125; d2r=pi/180;
wn=1.0; ze=0.8;                 %% attitude-regulator bandwidth / damping
a_pitch = -wn^2*(alpha_deg*d2r) - 2*ze*wn*q;   %% drive alpha->0, damp q
a_roll  = -wn^2*(phi_rad)       - 2*ze*wn*p;   %% wings level
a_yaw   = -wn^2*(beta_deg*d2r)  - 2*ze*wn*r;   %% zero sideslip
My = Iyy*a_pitch;  Mx = Ixx*a_roll;  Mz = Izz*a_yaw;
MxM=50000; MyM=120000; MzM=120000;             %% RCS moment authority [N*m] (placeholder)
Mx=max(-MxM,min(MxM,Mx)); My=max(-MyM,min(MyM,My)); Mz=max(-MzM,min(MzM,Mz));
onH  = double(h > 15000.0);                    %% only active high (thin air)
fade = max(0.0, min(1.0, (6000.0 - qbar)/(6000.0-1000.0)));  %% fade out as qbar builds
g = onH*fade;
F6 = [0.0; 0.0; 0.0; g*Mx; g*My; g*Mz];        %% [Fx;Fy;Fz;Mx;My;Mz] body
end

== matlab function ACFT11_a_121_flatearth_backup/FCS/HeadingHold/L1law ==
  data: psi_cmd input; phi output; track input; V input; qbar input
function phi = L1law(psi_cmd, track, V, qbar)
%#codegen
% L1 lateral-acceleration guidance with qbar-dependent authority.
% At low qbar (high altitude), bank command is scaled down so the
% INDI does not saturate and stall the solver.
g = 9.80665;
L1_tc = 15.0;
Vs = max(V, 30.0);
eta = (psi_cmd - track) * pi/180;
eta_w = atan2(sin(eta), cos(eta));
if abs(eta_w) > pi/2
    s = sign(eta_w);
    if s == 0, s = 1; end
    a_lat = s * (2.0*Vs/L1_tc);
else
    a_lat = (2.0*Vs/L1_tc) * sin(eta_w);
end
phi_raw = atan2(a_lat, g) * 180.0/pi;
qbar_scale = min(1.0, max(0.05, qbar / 5000.0));
phi = phi_raw * qbar_scale;
end

== matlab function ACFT11_a_121_flatearth_backup/Traj3D ==
  data: N input; E input; alt input; phase input
function Traj3D(N, E, alt, phase)
    coder.extrinsic('traj3d_plot');
    traj3d_plot(N, E, alt, phase);
end

== matlab function ACFT11_a_121_flatearth_backup/GlideCompute ==
  data: h input; glide_gamma_cmd output; range_home input; bearing_home input; gs_alt_cmd input; glide_psi_cmd output; app_h_cmd output
function [glide_gamma_cmd, glide_psi_cmd, app_h_cmd] = GlideCompute(h, range_home, bearing_home, gs_alt_cmd)
%#codegen
h_relight = 10000.0;
gamma_shallow = 3.0;
gamma_steep = 18.0;
safe_range = range_home + 1000.0;
raw_gamma = atan2d(h - h_relight, safe_range);
mid = 0.5*(gamma_shallow + gamma_steep);
half = 0.5*(gamma_steep - gamma_shallow);
clamped = mid + half * (2/pi) * atan((raw_gamma - mid) / (half * 0.3));
glide_gamma_cmd = -clamped;
gate = 1.0 / (1.0 + exp((h - 19000.0) / 500.0));
glide_psi_cmd = bearing_home * gate;
h_flare = 20.0;
app_h_cmd = 0.5*(gs_alt_cmd + h_flare + sqrt((gs_alt_cmd - h_flare)^2 + 100.0));
end

== matlab function ACFT11_a_121_flatearth_backup/MassModel ==
  settings: updateMethod=DISCRETE  sampleTime=0.05
  data: fuel_burned input; mass_kg output; sep_cmd input; Inertia output
function [mass_kg, Inertia] = MassModel(fuel_burned, sep_cmd)
%#codegen
persistent separated
if isempty(separated), separated = false; end
if sep_cmd > 0.5, separated = true; end
M_full = 28500.0; M_orb = 3000.0; M_empty = 10800.0;
mass_kg = M_full - fuel_burned;
if separated, mass_kg = mass_kg - M_orb; end
if mass_kg < M_empty, mass_kg = M_empty; end
bp = [10800.0, 25500.0, 28500.0];
Ixx_t = [32379.0, 52000.0, 74848.0];
Iyy_t = [136386.0, 200000.0, 288344.0];
Izz_t = [168765.0, 268000.0, 390125.0];
Ixz_t = [2511.0, 1800.0, 2511.0];
m = mass_kg;
if m < bp(1), m = bp(1); end
if m > bp(3), m = bp(3); end
if m <= bp(2)
  f = (m - bp(1)) / (bp(2) - bp(1));
  ixx = Ixx_t(1)+f*(Ixx_t(2)-Ixx_t(1));
  iyy = Iyy_t(1)+f*(Iyy_t(2)-Iyy_t(1));
  izz = Izz_t(1)+f*(Izz_t(2)-Izz_t(1));
  ixz = Ixz_t(1)+f*(Ixz_t(2)-Ixz_t(1));
else
  f = (m - bp(2)) / (bp(3) - bp(2));
  ixx = Ixx_t(2)+f*(Ixx_t(3)-Ixx_t(2));
  iyy = Iyy_t(2)+f*(Iyy_t(3)-Iyy_t(2));
  izz = Izz_t(2)+f*(Izz_t(3)-Izz_t(2));
  ixz = Ixz_t(2)+f*(Ixz_t(3)-Ixz_t(2));
end
Inertia = [ixx 0 -ixz; 0 iyy 0; -ixz 0 izz];
end

== matlab function ACFT11_a_121_flatearth_backup/WindModels/MeanWind ==
  data: h input; W_ned output
function W_ned = MeanWind(h)
%#codegen
% Upper-level MEAN wind (jetstream) in NED [W_N;W_E;W_D] m/s. Low-alt mean+shear
% is handled by the Wind Shear block; this adds the jetstream aloft.
Wjet=35.0; h_jet=11000.0; sig=3500.0; dir_deg=270.0;
spd=Wjet*exp(-((h-h_jet)/sig)^2);
to_rad=(dir_deg+180.0)*pi/180.0;
W_ned=[spd*cos(to_rad); spd*sin(to_rad); 0.0];
end

== matlab function ACFT11_a_121_flatearth_backup/WindModels/Scheduler ==
  data: qbar input; g output; phase input; h input
function g = Scheduler(qbar, phase, h)
%#codegen
% g=[gTurb;gGust;gShear] in 0..1. Fade with qbar, cap above ~20 km, gust only
% in takeoff / transonic / approach-land phases.
qlo=200.0; qhi=5000.0;
fq=(qbar-qlo)/(qhi-qlo); if fq<0, fq=0; elseif fq>1, fq=1; end
fa=(20000.0-h)/5000.0; if fa<0, fa=0; elseif fa>1, fa=1; end
base=fq*fa;
on_gust=(phase>=1 && phase<=4) || (phase>=6 && phase<=7) || (phase>=13 && phase<=15);
g=[base; base*double(on_gust); base];
end
